simulink model "scheme_L2"  (R2023a)
settings: Solver=VariableStepAuto  StartTime=0.0  StopTime=10  MaxStep=0.01  RelTol=1e-3
settings Model: Creator=mrlin  LastModifiedBy=mrlin

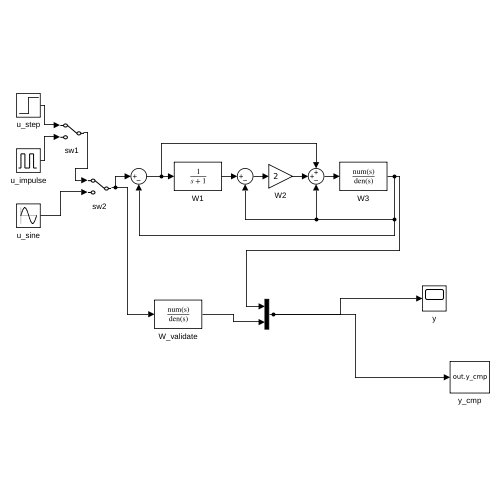
[thumbnail: Simulink's stored preview of the top-level diagram]
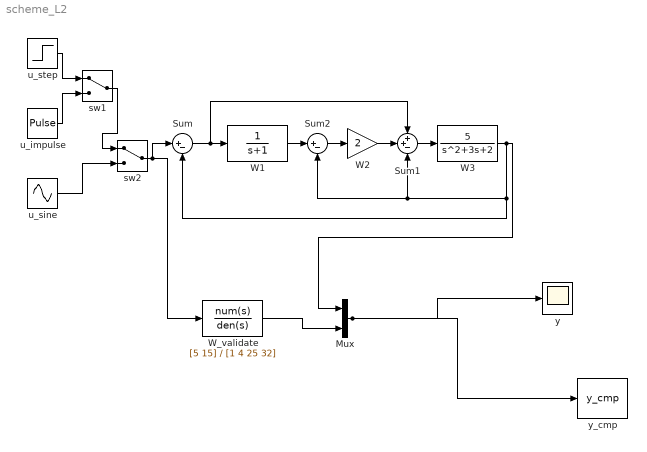
== system scheme_L2 ==
  Mux : Mux  Inputs=2
  Sum : Sum  Inputs=|+-
  Sum1 : Sum  Inputs=++-
  Sum2 : Sum  Inputs=|+-
  W1 : TransferFcn  Denominator=[1 1]
  W2 : Gain  Gain=2
  W3 : TransferFcn  Numerator=[5]  Denominator=[1 3 2]
  W_validate : TransferFcn  Numerator=[5 15]  Denominator=[1 4 25 32]
  sw1 : ManualSwitch
  sw2 : ManualSwitch
  u_impulse : DiscretePulseGenerator  PulseType=Time based  Amplitude=100  Period=100  PulseWidth=0.01
  u_sine : Sin  SampleTime=0
  u_step : Step  Time=0  SampleTime=0
  y : Scope
  y_cmp : ToWorkspace  VariableName=y_cmp  SaveFormat=Structure With Time  SampleTime=-1
  wires:
  Sum/1 -> Sum1/1, W1/1
  W1/1 -> Sum2/1
  Sum2/1 -> W2/1
  W2/1 -> Sum1/2
  Sum1/1 -> W3/1
  W3/1 -> Sum/2, Sum1/3, Sum2/2, Mux/1
  W_validate/1 -> Mux/2
  u_step/1 -> sw1/1
  u_impulse/1 -> sw1/2
  sw1/1 -> sw2/1
  u_sine/1 -> sw2/2
  sw2/1 -> Sum/1, W_validate/1
  Mux/1 -> y_cmp/1, y/1
